simulink model "QD2_DroneStack_PID_2021a"  (R2022a)
settings: Solver=ode1  StartTime=0.0  StopTime=inf  FixedStep=1/1000  RelTol=1e-3  EnableMultiTasking=on
InitFcn:
  | Motor_Mapping_7_Inch
model workspace (MAT data in the model file):
  target_system = 1
values from neighbouring files (symbols this model uses):
  KT = [0.03616,0.117,-0.01215]    [Motor_Mapping_7_Inch.m]
  Motor_Matrix = [ 0.25   -1/(2*L_Roll)    1/(2*L_Pitch)    K_Tau/4;                  0.25   -1/(2*L_Roll)   -1/(2*L_Pitch)   -K_Tau/4;                  0.25    1/(2*L_Roll)    1/(2*L_Pitch)   -K_Tau/4;                  0.25    1/(2*L_Roll)   -1/(2*L_Pitch)    K_Tau/4]    [Motor_Mapping_7_Inch.m]
undefined symbols (not defined in the file or in its folder): _Commander, _QDrone2, _Stabilizer, datetime, HIL, lf, log_, m, n, qc_get_step_size, s, saved_data
libraries: quarc_library x94, simulink x27, simulink_extras x9
(part 2 of 4)

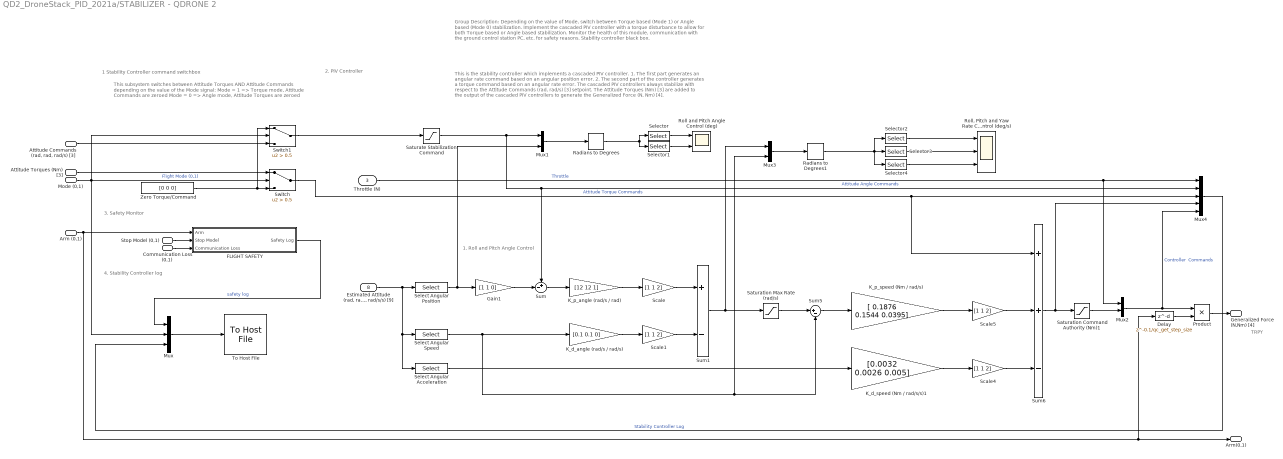
== system QD2_DroneStack_PID_2021a/STABILIZER - QDRONE 2 ==
  note: 3. Safety Monitor
  note: This subsystem switches between Attitude Torques AND Attitude Commands depending on
      | the value of the Mode signal:
      | Mode = 1	=> 		Torque mode, Attitude Commands are zeroed
      | Mode = 0	=> 		Angle mode, Attitude Torques are zeroed
  note: This is the stability controller which implements a cascaded PIV controller.
      | 1. The first part generates an angular rate command based on an angular position error.
      | 2. The second part of the controller generates a torque command based on an angular rate error.
      |
      | The cascaded PIV controllers always stabilize with respect to the Attitude Commands (rad, rad/s) [3] setpoint. The Attitude Torques (Nm) [3] are added to the output of the cascaded PIV controllers to generate the Generalized Force (N, Nm) [4].
  note: 1. Roll and Pitch Angle Control
  note: TRPY
  note: Group Description:
      |
      | Depending on the value of Mode, switch between Torque based (Mode 1) or Angle based (Mode 0) stabilization.
      | Implement the cascaded PIV controller with a torque disturbance to allow for both Torque based or Angle based stabilization.
      | Monitor the health of this module, communication with the ground control station PC, etc. for safety reasons.
      | Stability controller black box.
  note: 1 Stability Controller command switchbox
  note: 4. Stability Controller log
  note: 2. PIV Controller
  Mode (0,1) : Inport
  Stop Model (0,1) : Inport  Port=2
  Throttle (N) : Inport  Port=3
  Attitude Torques (Nm) [3] : Inport  Port=4
  "Attitude Commands (rad, rad, rad/s) [3]" : Inport  Port=5
  Arm (0,1) : Inport  Port=6
  Communication Loss (0,1) : Inport  Port=7
  "Estimated Attitude (rad, rad/s, rad/s/s) [9]" : Inport  Port=8
  Delay : Delay  DelayLength=0.1/qc_get_step_size
  FLIGHT SAFETY : Subsystem
  Gain1 : Gain  Gain=[1 1 0]
  K_d_angle (rad/s / rad/s) : Gain  Gain=[0.1 0.1 0]
  K_d_speed (Nm / rad/s/s)1 : Gain  Gain="[0.0032    0.0026     0.005]"
  K_p_angle (rad/s / rad) : Gain  Gain=[12 12 1]
  K_p_speed (Nm / rad/s) : Gain  Gain="[ 0.1876    0.1544    0.0395]"
  Mux : Mux  Inputs=3
  Mux1 : Mux  Inputs=2
  Mux2 : Mux  Inputs=2
  Mux3 : Mux  Inputs=2
  Mux4 : Mux  Inputs=5
  Product : Product
  Radians to Degrees : simulink_extras/Transformations/Radians to Degrees
  Radians to Degrees1 : simulink_extras/Transformations/Radians to Degrees
  Roll and Pitch Angle Control (deg) : Scope  NumInputPorts=2
  "Roll, Pitch and Yaw Rate Control (deg/s)" : Scope  NumInputPorts=3
  Saturate Stabilization Command : Saturate  UpperLimit=[pi/4 pi/4 10*pi/18]  LowerLimit=[-pi/4 -pi/4 -10*pi/18]
  Saturation Command Authority (Nm)1 : Saturate  UpperLimit=[1.0915 0.8984 0.0984]  LowerLimit=-[1.0915 0.8984 0.0984]
  Saturation Max Rate (rad/s) : Saturate  UpperLimit=10*pi/3*[1 1 1]  LowerLimit=-10*pi/3*[1 1 1]
  Scale{,1,4..5} (4 alike) : Gain  Gain=[1 1 2]
  Select Angular Acceleration : Selector  InputPortWidth=9  IndexOptions=Index vector (dialog)  Indices=[7:9]  OutputSizes=1
  Select Angular Speed : Selector  InputPortWidth=9  IndexOptions=Index vector (dialog)  Indices=[4:6]  OutputSizes=1
  Select Angular Position : Selector  InputPortWidth=9  IndexOptions=Index vector (dialog)  Indices=[1:3]  OutputSizes=1
  Selector : Selector  InputPortWidth=6  IndexOptions=Index vector (dialog)  Indices=[1 4]  OutputSizes=1
  Selector1 : Selector  InputPortWidth=6  IndexOptions=Index vector (dialog)  Indices=[2 5]  OutputSizes=1
  Selector2 : Selector  InputPortWidth=6  IndexOptions=Index vector (dialog)  Indices=[1 4]  OutputSizes=1
  Selector3 : Selector  InputPortWidth=6  IndexOptions=Index vector (dialog)  Indices=[2 5]  OutputSizes=1
  Selector4 : Selector  InputPortWidth=6  IndexOptions=Index vector (dialog)  Indices=[3 6]  OutputSizes=1
  Sum : Sum  Inputs=+-|
  Sum1 : Sum  Inputs=+-
  Sum5 : Sum  Inputs=|+-
  Sum6 : Sum  Inputs=++-
  Switch : Switch  Criteria=u2 > Threshold  Threshold=0.5  SaturateOnIntegerOverflow=off  InputSameDT=off
  Switch1 : Switch  Criteria=u2 > Threshold  Threshold=0.5  SaturateOnIntegerOverflow=off  InputSameDT=off
  To Host File : quarc_library/Sinks/To Host/To Host File  file_name=saved_data/%m/log_%{regexprep(char(datetime),' ','_')}_Stabilizer.mat  variable_name=stabilizer_data  decimation=1  sample_time=-1  file_format=MAT-file v.5  options=No header or footer  append=off  final_file_name=saved_data/QD2_DroneStack_PID_2021a/log_20-Nov-2026_20-05-50_Stabilizer.mat  bitrate=2000000
  Zero Torque/Command : Constant  Value=[0 0 0]
  Generalized Force (N,Nm) [4] : Outport  VectorParamsAs1DForOutWhenUnconnected=off
  Arm(0,1) : Outport  Port=2  VectorParamsAs1DForOutWhenUnconnected=off
  wires:
  Scale1/1 -> Sum1/2
  Scale/1 -> Sum1/1
  Delay/1 -> Product/2
  Zero Torque/Command/1 -> Switch1/1, Switch/3
  Attitude Torques (Nm) [3]/1 -> Switch/1
  "Attitude Commands (rad, rad, rad/s) [3]"/1 -> Switch1/3
  Radians to Degrees/1 -> Selector1/1, Selector/1
  K_d_angle (rad/s / rad/s)/1 -> Scale1/1
  Selector2/1 -> "Roll, Pitch and Yaw Rate Control (deg/s)"/1
  Selector/1 -> Roll and Pitch Angle Control (deg)/1
  Select Angular Speed/1 -> Mux3/2, Sum5/2, K_d_angle (rad/s / rad/s)/1
  K_p_angle (rad/s / rad)/1 -> Scale/1
  Selector4/1 -> "Roll, Pitch and Yaw Rate Control (deg/s)"/3
  Switch1/1 -> Saturate Stabilization Command/1
  Gain1/1 -> Sum/2
  Selector3/1 -> "Roll, Pitch and Yaw Rate Control (deg/s)"/2
  Mux1/1 -> Radians to Degrees/1
  "Estimated Attitude (rad, rad/s, rad/s/s) [9]"/1 -> Select Angular Speed/1, Select Angular Acceleration/1, Select Angular Position/1
  Radians to Degrees1/1 -> Selector3/1, Selector4/1, Selector2/1
  Switch/1 -> Sum6/1, Mux4/3  "Attitude Torque Commands"
  Selector1/1 -> Roll and Pitch Angle Control (deg)/2
  Throttle (N)/1 -> Mux4/1, Mux2/1  "Throttle"
  Select Angular Position/1 -> Mux1/2, Gain1/1
  Mux2/1 -> Product/1, Mux4/5  "Controller  Commands"
  Saturate Stabilization Command/1 -> Mux4/2, Sum/1, Mux1/1  "Attitude Angle Commands"
  Sum1/1 -> Mux3/1, Saturation Max Rate (rad/s)/1
  Mux3/1 -> Radians to Degrees1/1
  Arm (0,1)/1 -> FLIGHT SAFETY/1(Arm), Delay/1, Arm(0,1)/1
  Sum/1 -> K_p_angle (rad/s / rad)/1
  FLIGHT SAFETY/1(Safety Log) -> Mux/1  "safety log"
  Mode (0,1)/1 -> Mux/2, Switch1/2, Switch/2  "Flight Mode (0,1)"
  Mux4/1 -> Mux/3  "Stability Controller Log"
  Mux/1 -> To Host File/1
  Communication Loss (0,1)/1 -> FLIGHT SAFETY/3(Communication Loss)
  Stop Model (0,1)/1 -> FLIGHT SAFETY/2(Stop Model)
  Product/1 -> Generalized Force (N,Nm) [4]/1
  Saturation Max Rate (rad/s)/1 -> Sum5/1
  Sum5/1 -> K_p_speed (Nm / rad/s)/1
  K_p_speed (Nm / rad/s)/1 -> Scale5/1
  K_d_speed (Nm / rad/s/s)1/1 -> Scale4/1
  Scale4/1 -> Sum6/3
  Select Angular Acceleration/1 -> K_d_speed (Nm / rad/s/s)1/1
  Sum6/1 -> Mux4/4, Saturation Command Authority (Nm)1/1
  Saturation Command Authority (Nm)1/1 -> Mux2/2
  Scale5/1 -> Sum6/2

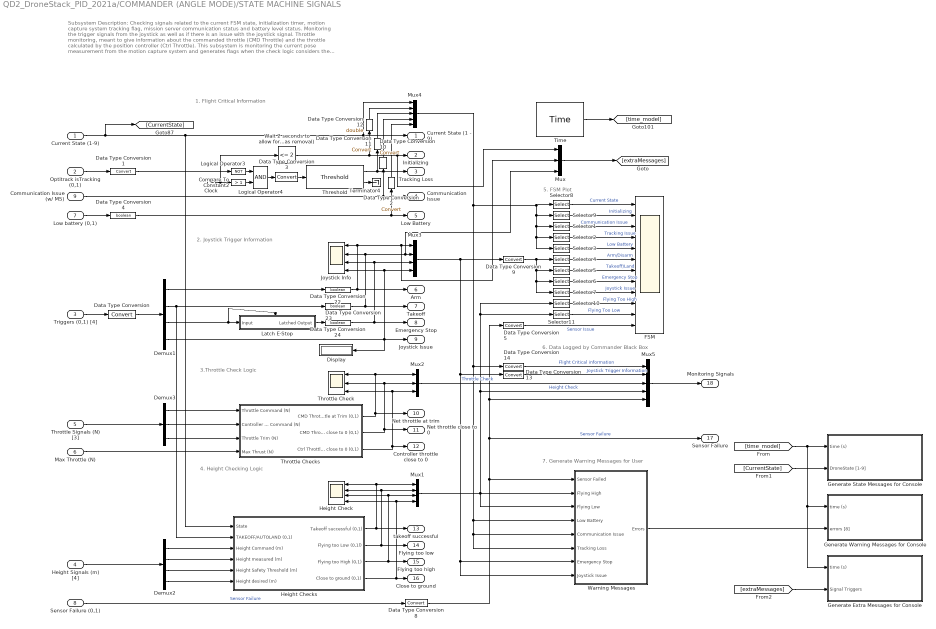
== system QD2_DroneStack_PID_2021a/COMMANDER (ANGLE MODE)/STATE MACHINE SIGNALS ==
  note: Subsystem Description:
      | Checking signals related to the current FSM state, initialization timer, motion capture system tracking flag, mission server communication status and battery level status.
      | Monitoring the trigger signals from the joystick as well as if there is an issue with the joystick signal.
      | Throttle monitoring, meant to give information about the commanded throttle (CMD Throttle) and the throttle calculated by the position controller (Ctrl Throttle).
      | This subsystem is monitoring the current pose measurement from the motion capture system and generates flags when the check logic considers the QDrone flying to close to ground, too high or too low as well as generate a successful take off flag.
      | A subset of the FSM monitoring signals are shown using this scope. These signals are what Quanser considers importnat for flight.
      | FSM signals sent to the blackbox for post flight monitoring.
      | Error message generation based on flags generated by the FSM signal checks.
  note: 7. Generate Warning Messages for User
  note: 5. FSM Plot
  note: 6. Data Logged by Commander Black Box
  note: 1. Flight Critical Information
  note: 2. Joystick Trigger Information
  note: 3.Throttle Check Logic
  note: 4. Height Checking Logic
  Current State (1-9) : Inport
  "Optitrack isTracking (0,1)  " : Inport  Port=2
  Triggers (0,1) [4] : Inport  Port=3
  Height Signals (m) [4] : Inport  Port=4
  Throttle Signals (N) [3] : Inport  Port=5
  "Max Throttle (N) " : Inport  Port=6
  Low battery (0,1) : Inport  Port=7
  Sensor Failure (0,1) : Inport  Port=8
  Communication Issue (w/ MS) : Inport  Port=9
  Clock : Clock
  Compare To Constant2 : simulink/Logic and Bit Operations/Compare To Constant  relop=>  const=1  OutDataTypeStr=boolean
  Data Type Conversion{,1..3,5,8..11,13..14} (11 alike) : DataTypeConversion  SaturateOnIntegerOverflow=off  RndMeth=Floor
  Data Type Conversion12 : DataTypeConversion  OutDataTypeStr=double  SaturateOnIntegerOverflow=off  RndMeth=Floor
  Data Type Conversion{4,22..24} (4 alike) : DataTypeConversion  OutDataTypeStr=boolean  SaturateOnIntegerOverflow=off  RndMeth=Floor
  Demux1 : Demux  Outputs=[1 1 1 1]
  Demux2 : Demux
  Demux3 : Demux  Outputs=3
  Display : Display
  FSM : Scope  NumInputPorts=12
  Generate Extra Messages for Console : Subsystem
  Generate State Messages for Console : Subsystem
  Generate Warning Messages for Console : Subsystem
  "Height Check " : Scope  NumInputPorts=4
  Height Checks : Subsystem
  Joystick Info : Scope  NumInputPorts=4
  Latch E-Stop : Subsystem  TreatAsAtomicUnit=on
  Logical Operator3 : Logic  Operator=NOT  AllPortsSameDT=off  OutDataTypeStr=boolean
  Logical Operator4 : Logic  AllPortsSameDT=off  OutDataTypeStr=boolean
  Mux : Mux  Inputs=3
  Mux1 : Mux  Inputs=[1 1 1 1]
  Mux2 : Mux  Inputs=[1 1 1]
  Mux3 : Mux  Inputs=[1 1 1 1]
  Mux4 : Mux  Inputs=[1 1 1 1 1]
  Mux5 : Mux  Inputs=[5 4 3 4 1]
  Selector1 : Selector  InputPortWidth=5  IndexOptions=Index vector (dialog)  Indices=4  OutputSizes=1
  Selector10 : Selector  InputPortWidth=4  IndexOptions=Index vector (dialog)  Indices=3  OutputSizes=1
  Selector11 : Selector  InputPortWidth=4  IndexOptions=Index vector (dialog)  Indices=2  OutputSizes=1
  Selector2 : Selector  InputPortWidth=5  IndexOptions=Index vector (dialog)  Indices=3  OutputSizes=1
  Selector3 : Selector  InputPortWidth=5  IndexOptions=Index vector (dialog)  Indices=5  OutputSizes=1
  Selector4 : Selector  InputPortWidth=4  IndexOptions=Index vector (dialog)  Indices=1  OutputSizes=1
  Selector5 : Selector  InputPortWidth=4  IndexOptions=Index vector (dialog)  Indices=2  OutputSizes=1
  Selector6 : Selector  InputPortWidth=4  IndexOptions=Index vector (dialog)  Indices=3  OutputSizes=1
  Selector7 : Selector  InputPortWidth=4  IndexOptions=Index vector (dialog)  Indices=4  OutputSizes=1
  Selector8 : Selector  InputPortWidth=5  IndexOptions=Index vector (dialog)  Indices=1  OutputSizes=1
  Selector9 : Selector  InputPortWidth=5  IndexOptions=Index vector (dialog)  Indices=2  OutputSizes=1
  Terminator4 : Terminator
  Threshold : quarc_library/Discontinuities/Threshold  operator=>=  param_src=Specify via dialog  threshold=0.5  duration=0.2
      settings: SourceProductName=QUARC Targets
  Throttle Check : Scope  NumInputPorts=3
  Throttle Checks : Subsystem
  Time : quarc_library/Sources/Time/Time  time_source=Wall clock  sample_time=qc_get_step_size
  "Wait 2 seconds to allow for initialization (e.g., bias removal)" : simulink/Logic and Bit Operations/Compare To Constant  relop=<=  const=2  OutDataTypeStr=boolean
  Warning Messages : Subsystem
  "Current State (1 - 9)  " : Outport  VectorParamsAs1DForOutWhenUnconnected=off
  Initializing : Outport  Port=2  VectorParamsAs1DForOutWhenUnconnected=off
  Tracking Loss : Outport  Port=3  VectorParamsAs1DForOutWhenUnconnected=off
  Communication Issue : Outport  Port=4  VectorParamsAs1DForOutWhenUnconnected=off
  Low Battery : Outport  Port=5  VectorParamsAs1DForOutWhenUnconnected=off
  Arm : Outport  Port=6  VectorParamsAs1DForOutWhenUnconnected=off
  Takeoff : Outport  Port=7  VectorParamsAs1DForOutWhenUnconnected=off
  Emergency Stop : Outport  Port=8  VectorParamsAs1DForOutWhenUnconnected=off
  "Joystick Issue " : Outport  Port=9  VectorParamsAs1DForOutWhenUnconnected=off
  Net throttle at trim : Outport  Port=10  VectorParamsAs1DForOutWhenUnconnected=off
  Net throttle close to 0 : Outport  Port=11  VectorParamsAs1DForOutWhenUnconnected=off
  Controller throttle close to 0 : Outport  Port=12  VectorParamsAs1DForOutWhenUnconnected=off
  takeoff successful : Outport  Port=13  VectorParamsAs1DForOutWhenUnconnected=off
  Flying too low : Outport  Port=14  VectorParamsAs1DForOutWhenUnconnected=off
  Flying too high : Outport  Port=15  VectorParamsAs1DForOutWhenUnconnected=off
  Close to ground : Outport  Port=16  VectorParamsAs1DForOutWhenUnconnected=off
  "  Sensor Failure" : Outport  Port=17  VectorParamsAs1DForOutWhenUnconnected=off
  Monitoring Signals : Outport  Port=18  VectorParamsAs1DForOutWhenUnconnected=off
  wires:
  Triggers (0,1) [4]/1 -> Data Type Conversion/1
  Demux2/1 -> Height Checks/3(Height Command (m))
  Demux3/1 -> Throttle Checks/1(Throttle Command (N))
  Height Signals (m) [4]/1 -> Demux2/1
  Demux2/4 -> Height Checks/6(Height desired (m))
  Throttle Signals (N) [3]/1 -> Demux3/1
  Demux1/1 -> Data Type Conversion22/1
  Throttle Checks/2(CMD Throttle close to 0 (0,1)) -> Mux2/2, Throttle Check/2, Net throttle close to 0/1
  Height Checks/1(Takeoff successful (0,1)) -> takeoff successful/1, "Height Check "/1, Mux1/1
  Demux2/3 -> Height Checks/5(Height Safety Threshold (m))
  Demux1/2 -> Data Type Conversion23/1, Height Checks/2(TAKEOFF/AUTOLAND (0,1))
  Demux2/2 -> Height Checks/4(Height measured (m))
  Demux3/2 -> Throttle Checks/2(Controller Throttle Command (N))
  Demux3/3 -> Throttle Checks/3(Throttle Trim (N))
  Throttle Checks/1(CMD Throttle at Trim (0,1)) -> Net throttle at trim/1, Mux2/1, Throttle Check/1
  Height Checks/3(Flying too High (0,1)) -> Mux1/3, "Height Check "/3, Flying too high/1
  Height Checks/4(Close to ground (0,1)) -> "Height Check "/4, Mux1/4, Close to ground/1
  Data Type Conversion/1 -> Demux1/1
  Low battery (0,1)/1 -> Data Type Conversion4/1
  Height Checks/2(Flying too Low (0,1l)) -> Flying too low/1, Mux1/2, "Height Check "/2
  Sensor Failure (0,1)/1 -> Data Type Conversion8/1  "Sensor Failure"
  Data Type Conversion1/1 -> Logical Operator3/1
  Data Type Conversion3/1 -> Threshold/1
  Compare To Constant2/1 -> Logical Operator4/2
  Clock/1 -> "Wait 2 seconds to allow for initialization (e.g., bias removal)"/1, Compare To Constant2/1
  Logical Operator4/1 -> Data Type Conversion3/1
  Threshold/2 -> Terminator4/1
  Logical Operator3/1 -> Logical Operator4/1
  "Optitrack isTracking (0,1)  "/1 -> Data Type Conversion1/1
  Latch E-Stop/1(Latched Output) -> Data Type Conversion24/1
  Demux1/3 -> Latch E-Stop/1(Input), Latch E-Stop/Trigger
  Selector9/1 -> FSM/2  "Initializing"
  Selector1/1 -> FSM/3  "Communication Issue"
  Selector2/1 -> FSM/4  "Tracking Issue"
  Selector3/1 -> FSM/5  "Low Battery"
  Selector4/1 -> FSM/6  "Arm/Disarm"
  Selector5/1 -> FSM/7  "Takeoff/Land"
  Selector6/1 -> FSM/8  "Emergency Stop"
  Selector7/1 -> FSM/9  "Joystick Issue"
  Data Type Conversion5/1 -> FSM/12  "Sensor Issue"
  Selector10/1 -> FSM/10  "Flying Too High"
  Selector11/1 -> FSM/11  "Flying Too Low"
  Data Type Conversion24/1 -> Joystick Info/3, Mux3/3, Emergency Stop/1
  Data Type Conversion23/1 -> Joystick Info/2, Mux/3, Mux3/2, Takeoff/1
  Data Type Conversion22/1 -> Joystick Info/1, Mux/2, Mux3/1, Arm/1
  Data Type Conversion4/1 -> Low Battery/1, Data Type Conversion2/1
  Demux1/4 -> Display/1, Joystick Info/4, Mux3/4, "Joystick Issue "/1
  Communication Issue (w/ MS)/1 -> Communication Issue/1, Data Type Conversion10/1
  Threshold/1 -> Tracking Loss/1, Data Type Conversion11/1
  Mux5/1 -> Monitoring Signals/1
  Mux1/1 -> Warning Messages/3(Flying Low), Warning Messages/2(Flying High), Selector11/1, Selector10/1, Mux5/4  "Height Check"
  Mux2/1 -> Mux5/3  "Throttle Check"
  Mux3/1 -> Data Type Conversion9/1, Warning Messages/7("Emergency Stop "), Warning Messages/8(Joystick Issue), Data Type Conversion13/1
  Mux4/1 -> Warning Messages/4(Low Battery), Warning Messages/5(Communication Issue), Warning Messages/6(Tracking Loss), Data Type Conversion14/1, Selector3/1, Selector2/1, Selector1/1, Selector9/1, Selector8/1
  Throttle Checks/3(Ctrl Throttle close to 0 (0,1)) -> Mux2/3, Throttle Check/3, Controller throttle close to 0/1
  Data Type Conversion9/1 -> Selector4/1, Selector5/1, Selector7/1, Selector6/1
  Data Type Conversion8/1 -> "  Sensor Failure"/1, Data Type Conversion5/1, Mux5/5, Warning Messages/1(Sensor Failed)  "Sensor Failure"
  Current State (1-9)/1 -> [CurrentState], Mux4/1, "Current State (1 - 9)  "/1, Height Checks/1(State)
  Selector8/1 -> FSM/1  "Current State"
  Data Type Conversion2/1 -> Mux4/5
  Data Type Conversion10/1 -> Mux4/4
  Data Type Conversion11/1 -> Mux4/3
  Data Type Conversion12/1 -> Mux4/2
  Data Type Conversion13/1 -> Mux5/2  "Joystick Trigger Information"
  Data Type Conversion14/1 -> Mux5/1  "Flight Critical information"
  "Wait 2 seconds to allow for initialization (e.g., bias removal)"/1 -> Data Type Conversion12/1, Mux/1, Initializing/1
  "Max Throttle (N) "/1 -> Throttle Checks/4(Max Thrust (N))
  Time/1 -> [time_model]
  [time_model] -> Generate Warning Messages for Console/1(time (s)), Generate Extra Messages for Console/1(time (s)), Generate State Messages for Console/1(time (s))
  [CurrentState] -> Generate State Messages for Console/2(DroneState [1-9])
  Warning Messages/1(Errors) -> Generate Warning Messages for Console/2(errors [8])
  Mux/1 -> [extraMessages]
  [extraMessages] -> Generate Extra Messages for Console/2(Signal Triggers)

== system QD2_DroneStack_PID_2021a/COMMANDER (ANGLE MODE)/Signal Smoothing ==
  "High Frequency Controller Commands (N,rad, rad/s)[4]" : Inport
  Constant4 : Constant
  Constant5 : Constant  Value=100
  Mux : Mux  Inputs=2
  Second-Order Low-Pass Filter : quarc_library/Continuous/Second-Order Low-Pass Filter  params_source=External (input ports)  input_width=60  input_zeta=1  input_init=0
  Selector1 : Selector  InputPortWidth=4  IndexOptions=Index vector (dialog)  Indices=[3:4]  OutputSizes=1
  Selector3 : Selector  InputPortWidth=4  IndexOptions=Index vector (dialog)  Indices=[1:2]  OutputSizes=1
  Terminator : Terminator
  "Smoothed Controller Commands (N,rad, rad/s)[4]" : Outport
  wires:
  "High Frequency Controller Commands (N,rad, rad/s)[4]"/1 -> Selector1/1, Selector3/1
  Mux/1 -> "Smoothed Controller Commands (N,rad, rad/s)[4]"/1
  Selector1/1 -> Mux/2
  Second-Order Low-Pass Filter/1 -> Mux/1
  Selector3/1 -> Second-Order Low-Pass Filter/4, Second-Order Low-Pass Filter/1
  Constant4/1 -> Second-Order Low-Pass Filter/3
  Constant5/1 -> Second-Order Low-Pass Filter/2
  Second-Order Low-Pass Filter/2 -> Terminator/1

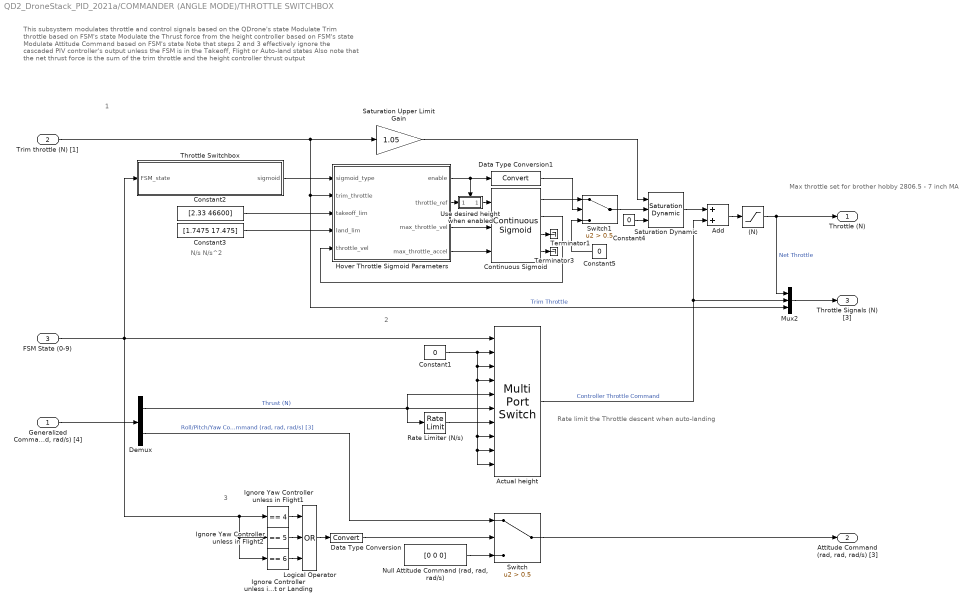
== system QD2_DroneStack_PID_2021a/COMMANDER (ANGLE MODE)/THROTTLE SWITCHBOX  ==
  note: Max throttle set for brother hobby 2806.5 - 7 inch MA
  note: 3
  note: 2
  note: 1
  note: Rate limit the Throttle descent when auto-landing
  note: This subsystem modulates throttle and control signals based on the QDrone's state
      | Modulate Trim throttle based on FSM's state
      | Modulate the Thrust force from the height controller based on FSM's state
      | Modulate Attitude Command based on FSM's state
      |
      | Note that steps 2 and 3 effectively ignore the cascaded PIV controller's output unless the FSM is in the Takeoff, Flight or Auto-land states
      | Also note that the net thrust force is the sum of the trim throttle and the height controller thrust output
  note: N/s N/s^2
  "Generalized Command (N, rad, rad, rad/s) [4]" : Inport
  Trim throttle (N) [1] : Inport  Port=2
  FSM State (0-9) : Inport  Port=3
  (N) : Saturate  UpperLimit=58  LowerLimit=0
  Actual height : MultiPortSwitch  Inputs=9  SaturateOnIntegerOverflow=off  InputSameDT=off
  Add : Sum
  Constant1 : Constant  Value=0
  Constant2 : Constant  Value=[2.33 46600]
  Constant3 : Constant  Value=[1.7475 17.475]
  Constant4 : Constant  Value=0
  Constant5 : Constant  Value=0
  Continuous Sigmoid : quarc_library/Sources/Sigmoids/Continuous Sigmoid  params_source=External (input ports)  max_velocity=2  max_acceleration=10  initial_position=0  initial_velocity=0  hold_off=0.5  input_sample_time=-1  output_sample_time=qc_get_step_size
      settings: SourceProductName=QUARC Targets
  Data Type Conversion : DataTypeConversion  SaturateOnIntegerOverflow=off  RndMeth=Floor
  Data Type Conversion1 : DataTypeConversion  SaturateOnIntegerOverflow=off  RndMeth=Floor
  Demux : Demux  Outputs=[1 3]
  Hover Throttle Sigmoid Parameters : MATLAB Function  TreatAsAtomicUnit=on
  "Ignore Controller unless in Takeoff, Flight or Landing" : simulink/Logic and Bit Operations/Compare To Constant  relop===  const=6  OutDataTypeStr=boolean
  Ignore Yaw Controller unless in Flight1 : simulink/Logic and Bit Operations/Compare To Constant  relop===  const=4  OutDataTypeStr=boolean
  Ignore Yaw Controller unless in Flight2 : simulink/Logic and Bit Operations/Compare To Constant  relop===  const=5  OutDataTypeStr=boolean
  Logical Operator : Logic  Operator=OR  Inputs=3  AllPortsSameDT=off  OutDataTypeStr=boolean
  Mux2 : Mux  Inputs=3
  "Null Attitude Command (rad, rad, rad/s)" : Constant  Value=[0 0 0]
  Rate Limiter (N/s) : RateLimiter  RisingSlewLimit=100  FallingSlewLimit=-100  SampleTimeMode=inherited
  Saturation Dynamic : simulink/Discontinuities/Saturation Dynamic  OutMin=[]  OutMax=[]  OutDataTypeStr=Inherit: Same as second input  OutDataType=fixdt(1, 16)  OutScaling=2^-10  DoSatur=off
  Saturation Upper Limit Gain : Gain  Gain=1.05
  Switch : Switch  Criteria=u2 > Threshold  Threshold=0.5  SaturateOnIntegerOverflow=off  InputSameDT=off
  Switch1 : Switch  Criteria=u2 > Threshold  Threshold=0.5  SaturateOnIntegerOverflow=off  InputSameDT=off
  Terminator1 : Terminator
  Terminator3 : Terminator
  Throttle Switchbox : MATLAB Function  TreatAsAtomicUnit=on
  Use desired height when enabled : Subsystem  TreatAsAtomicUnit=on
  Throttle (N) : Outport  VectorParamsAs1DForOutWhenUnconnected=off
  "Attitude Command (rad, rad, rad/s) [3]" : Outport  Port=2  VectorParamsAs1DForOutWhenUnconnected=off
  Throttle Signals (N) [3] : Outport  Port=3  VectorParamsAs1DForOutWhenUnconnected=off
  wires:
  Actual height/1 -> Mux2/2, Add/2  "Controller Throttle Command"
  Add/1 -> (N)/1
  (N)/1 -> Mux2/1, Throttle (N)/1  "Net Throttle"
  "Generalized Command (N, rad, rad, rad/s) [4]"/1 -> Demux/1
  Mux2/1 -> Throttle Signals (N) [3]/1
  Ignore Yaw Controller unless in Flight2/1 -> Logical Operator/2
  Data Type Conversion/1 -> Switch/2
  "Null Attitude Command (rad, rad, rad/s)"/1 -> Switch/3
  Ignore Yaw Controller unless in Flight1/1 -> Logical Operator/1
  Demux/2 -> Switch/1  "Roll/Pitch/Yaw Command (rad, rad, rad/s) [3]"
  FSM State (0-9)/1 -> Actual height/1, "Ignore Controller unless in Takeoff, Flight or Landing"/1, Ignore Yaw Controller unless in Flight2/1, Ignore Yaw Controller unless in Flight1/1, Throttle Switchbox/1(FSM_state)
  "Ignore Controller unless in Takeoff, Flight or Landing"/1 -> Logical Operator/3
  Logical Operator/1 -> Data Type Conversion/1
  Demux/1 -> Actual height/6, Rate Limiter (N/s)/1, Actual height/5  "Thrust (N)"
  Continuous Sigmoid/2 -> Hover Throttle Sigmoid Parameters/5(throttle_vel)
  Constant4/1 -> Saturation Dynamic/3
  Saturation Dynamic/1 -> Add/1
  Constant3/1 -> Hover Throttle Sigmoid Parameters/4(land_lim)
  Switch1/1 -> Saturation Dynamic/2
  Trim throttle (N) [1]/1 -> Mux2/3, Hover Throttle Sigmoid Parameters/2(trim_throttle), Saturation Upper Limit Gain/1  "Trim Throttle"
  Throttle Switchbox/1(sigmoid) -> Hover Throttle Sigmoid Parameters/1(sigmoid_type)
  Saturation Upper Limit Gain/1 -> Saturation Dynamic/1
  Constant2/1 -> Hover Throttle Sigmoid Parameters/3(takeoff_lim)
  Hover Throttle Sigmoid Parameters/4(max_throttle_accel) -> Continuous Sigmoid/3
  Continuous Sigmoid/1 -> Switch1/1
  Continuous Sigmoid/4 -> Terminator3/1
  Hover Throttle Sigmoid Parameters/3(max_throttle_vel) -> Continuous Sigmoid/2
  Data Type Conversion1/1 -> Switch1/2
  Hover Throttle Sigmoid Parameters/1(enable) -> Data Type Conversion1/1, Use desired height when enabled/Enable
  Continuous Sigmoid/3 -> Terminator1/1
  Use desired height when enabled/1(Out1) -> Continuous Sigmoid/1
  Hover Throttle Sigmoid Parameters/2(throttle_ref) -> Use desired height when enabled/1(h_d (m) [1])
  Constant5/1 -> Switch1/3
  Switch/1 -> "Attitude Command (rad, rad, rad/s) [3]"/1
  Constant1/1 -> Actual height/8, Actual height/10, Actual height/9, Actual height/4, Actual height/3, Actual height/2
  Rate Limiter (N/s)/1 -> Actual height/7

== system QD2_DroneStack_PID_2021a/Communication/Detect Communication Loss ==
  note: Stream Loss: Check if the state is 2 and error is positive (error codes are negative). Otherwise issue a communication error.
      | OR
      | Data Loss: Check if the data is stale for a while (this is required because a connected stream may publish no new data). If stale, issue a communication error.
  State : Inport
  Error : Inport  Port=2
  Data Out : Inport  Port=3
  Clock1 : Clock
  Communication Loss : Scope  NumInputPorts=2
  Data Type Conversion4 : DataTypeConversion  SaturateOnIntegerOverflow=off  RndMeth=Floor
  Grab mission server time to detect flat lines : Selector  InputPortWidth=16  IndexOptions=Index vector (dialog)  Indices=[16]  OutputSizes=1
  Logical Operator4 : Logic  Operator=OR  AllPortsSameDT=off  OutDataTypeStr=boolean
  MATLAB Function : MATLAB Function  TreatAsAtomicUnit=on
  Terminator3 : Terminator
  Terminator5 : Terminator
  Threshold1 : quarc_library/Discontinuities/Threshold  operator=>=  param_src=Specify via dialog  threshold=0.5  duration=0.1
      settings: SourceProductName=QUARC Targets
  Threshold2 : quarc_library/Discontinuities/Threshold  operator=>=  param_src=Specify via dialog  threshold=0.5  duration=0.5
      settings: SourceProductName=QUARC Targets
  Communication Issue : Outport  VectorParamsAs1DForOutWhenUnconnected=off
  wires:
  Threshold2/1 -> Communication Loss/2, Logical Operator4/2
  Logical Operator4/1 -> Data Type Conversion4/1
  Threshold1/2 -> Terminator3/1
  MATLAB Function/2(data_loss) -> Threshold2/1
  MATLAB Function/1(stream_connection_loss) -> Threshold1/1
  Clock1/1 -> MATLAB Function/1(time)
  Threshold2/2 -> Terminator5/1
  Threshold1/1 -> Communication Loss/1, Logical Operator4/1
  Grab mission server time to detect flat lines/1 -> MATLAB Function/4(ms_time)
  Data Out/1 -> Grab mission server time to detect flat lines/1
  State/1 -> MATLAB Function/2(state)
  Error/1 -> MATLAB Function/3(error)
  Data Type Conversion4/1 -> Communication Issue/1

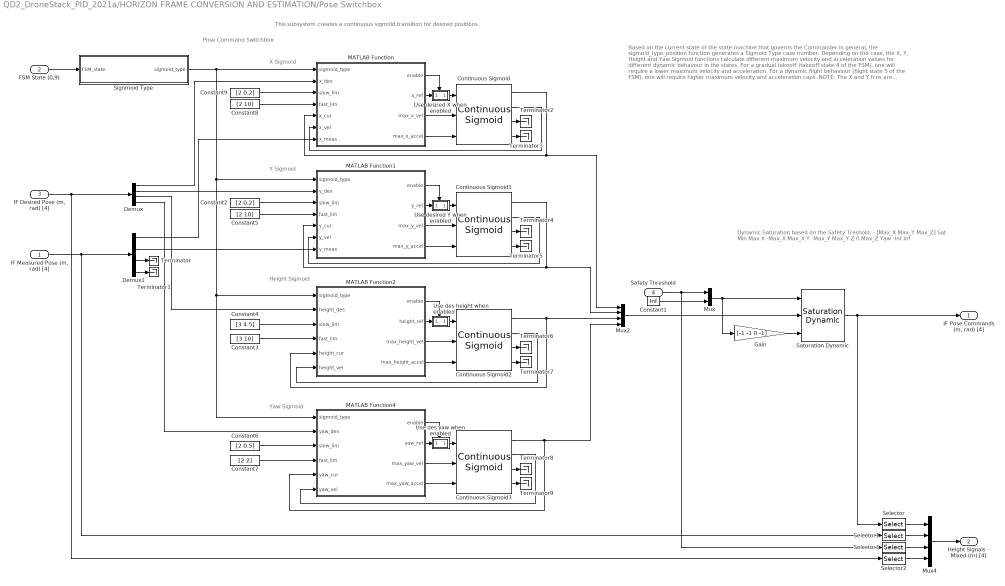
== system QD2_DroneStack_PID_2021a/HORIZON FRAME CONVERSION AND ESTIMATION/Pose Switchbox ==
  note: Dynamic Saturation based on the Safety Treshold. - [Max_X Max_Y Max_Z]
      |
      | Sat Min Max
      | X -Max_X Max_X
      | Y -Max_Y Max_Y
      | Z 0 Max_Z
      | Yaw -Inf Inf
  note: Based on the current state of the state machine that governs the Commander in general,
      | the sigmoid_type_position function generates a Sigmoid Type case number. Depending on
      | the case, the X, Y, Height and Yaw Sigmoid functions calculate different maximum velocity
      | and acceleration values for different dynamic behavour in the states.
      |
      | For a gradual takeoff (takeoff state 4 of the FSM), one will require a lower maximum velocity
      | and acceleration. For a dynamic flight behaviour (flight state 5 of the FSM), one will require
      | higher maximum velocity and acceleration caps.
      |
      | NOTE: The X and Y fcns are logically identical due to the generally symmetric X and Y behaviour.
      | The Z and Yaw fcns are different.
  note: This subsystem creates a continuous sigmoid transition for desired positions.
  note: Height Sigmoid
  note: Pose Command Switchbox
  note: X Sigmoid
  note: Yaw Sigmoid
  note: Y Sigmoid
  "IF Measured Pose (m, rad) [4]" : Inport
  FSM State (0,9) : Inport  Port=2
  "IF Desired Pose (m, rad) [4]" : Inport  Port=3
  Safety Threshold : Inport  Port=4
  Constant1 : Constant  Value=Inf
  Constant2 : Constant  Value=[2 0.2]
  Constant3 : Constant  Value=[3 10]
  Constant4 : Constant  Value=[3 4.5]
  Constant5 : Constant  Value=[2 10]
  Constant6 : Constant  Value=[2 0.5]
  Constant7 : Constant  Value=[2 2]
  Constant8 : Constant  Value=[2 10]
  Constant9 : Constant  Value=[2 0.2]
  Continuous Sigmoid{,1..3} (4 alike) : quarc_library/Sources/Sigmoids/Continuous Sigmoid  params_source=External (input ports)  max_velocity=2  max_acceleration=10  initial_position=0  initial_velocity=0  hold_off=0.5  input_sample_time=-1  output_sample_time=qc_get_step_size
      settings: SourceProductName=QUARC Targets
  Demux : Demux
  Demux1 : Demux
  Gain : Gain  Gain=[-1 -1 0 -1]
  MATLAB Function : MATLAB Function  TreatAsAtomicUnit=on
  MATLAB Function1 : MATLAB Function  TreatAsAtomicUnit=on
  MATLAB Function2 : MATLAB Function  TreatAsAtomicUnit=on
  MATLAB Function4 : MATLAB Function  TreatAsAtomicUnit=on
  Mux : Mux  Inputs=2
  Mux2 : Mux
  Mux4 : Mux
  Saturation Dynamic : simulink/Discontinuities/Saturation Dynamic  OutMin=[]  OutMax=[]  OutDataTypeStr=Inherit: Same as second input  OutDataType=fixdt(1, 16)  OutScaling=2^-10  DoSatur=off
  Selector : Selector  InputPortWidth=4  IndexOptions=Index vector (dialog)  Indices=[3]  OutputSizes=1
  Selector1 : Selector  InputPortWidth=4  IndexOptions=Index vector (dialog)  Indices=[3]  OutputSizes=1
  Selector2 : Selector  InputPortWidth=4  IndexOptions=Index vector (dialog)  Indices=[3]  OutputSizes=1
  Selector3 : Selector  InputPortWidth=3  IndexOptions=Index vector (dialog)  Indices=[3]  OutputSizes=1
  Signmoid Type : MATLAB Function  TreatAsAtomicUnit=on
  Terminator{,1..9} (10 alike) : Terminator
  Use des height when enabled : Subsystem  TreatAsAtomicUnit=on
  Use des yaw when enabled : Subsystem  TreatAsAtomicUnit=on
  Use desired X when enabled : Subsystem  TreatAsAtomicUnit=on
  Use desired Y when enabled : Subsystem  TreatAsAtomicUnit=on
  "IF Pose Commands (m, rad) [4]" : Outport  VectorParamsAs1DForOutWhenUnconnected=off
  Height Signals - Mixed (m) [4] : Outport  Port=2  VectorParamsAs1DForOutWhenUnconnected=off
  wires:
  Constant4/1 -> MATLAB Function2/3(slow_lim)
  Constant3/1 -> MATLAB Function2/4(fast_lim)
  Selector/1 -> Mux4/1
  Selector1/1 -> Mux4/2
  Selector2/1 -> Mux4/4
  Selector3/1 -> Mux4/3
  Safety Threshold/1 -> Mux/1, Selector3/1
  Mux/1 -> Saturation Dynamic/1, Gain/1
  Constant1/1 -> Mux/2
  Saturation Dynamic/1 -> "IF Pose Commands (m, rad) [4]"/1, Selector/1
  Mux2/1 -> Saturation Dynamic/2
  Mux4/1 -> Height Signals - Mixed (m) [4]/1
  Gain/1 -> Saturation Dynamic/3
  Demux/2 -> MATLAB Function1/2(y_des)
  Use desired Y when enabled/1(Out1) -> Continuous Sigmoid1/1
  Use desired X when enabled/1(Out1) -> Continuous Sigmoid/1
  MATLAB Function2/3(max_height_vel) -> Continuous Sigmoid2/2
  Continuous Sigmoid3/3 -> Terminator8/1
  Demux1/4 -> Terminator1/1
  MATLAB Function4/1(enable) -> Use des yaw when enabled/Enable
  Use des yaw when enabled/1(Out1) -> Continuous Sigmoid3/1
  Continuous Sigmoid1/2 -> MATLAB Function1/6(y_vel)
  Constant2/1 -> MATLAB Function1/3(slow_lim)
  Constant6/1 -> MATLAB Function4/3(slow_lim)
  Demux1/1 -> MATLAB Function/7(x_meas)
  MATLAB Function1/2(y_ref) -> Use desired Y when enabled/1(h_d (m) [1])
  Demux/3 -> MATLAB Function2/2(height_des)
  Constant7/1 -> MATLAB Function4/4(fast_lim)
  Continuous Sigmoid1/4 -> Terminator5/1
  MATLAB Function1/1(enable) -> Use desired Y when enabled/Enable
  Continuous Sigmoid2/4 -> Terminator7/1
  Demux1/3 -> Terminator/1
  Signmoid Type/1(sigmoid_type) -> MATLAB Function/1(sigmoid_type), MATLAB Function1/1(sigmoid_type), MATLAB Function2/1(sigmoid_type), MATLAB Function4/1(sigmoid_type)
  MATLAB Function/3(max_x_vel) -> Continuous Sigmoid/2
  MATLAB Function2/1(enable) -> Use des height when enabled/Enable
  Constant9/1 -> MATLAB Function/3(slow_lim)
  Continuous Sigmoid2/2 -> MATLAB Function2/6(height_vel)
  Continuous Sigmoid1/1 -> MATLAB Function1/5(y_cur), Mux2/2
  MATLAB Function4/4(max_yaw_accel) -> Continuous Sigmoid3/3
  Demux/1 -> MATLAB Function/2(x_des)
  MATLAB Function1/3(max_y_vel) -> Continuous Sigmoid1/2
  Continuous Sigmoid3/2 -> MATLAB Function4/6(yaw_vel)
  MATLAB Function2/2(height_ref) -> Use des height when enabled/1(h_d (m) [1])
  MATLAB Function/4(max_x_accel) -> Continuous Sigmoid/3
  Use des height when enabled/1(Out1) -> Continuous Sigmoid2/1
  Continuous Sigmoid2/3 -> Terminator6/1
  Demux/4 -> MATLAB Function4/2(yaw_des)
  MATLAB Function1/4(max_y_accel) -> Continuous Sigmoid1/3
  MATLAB Function/1(enable) -> Use desired X when enabled/Enable
  Continuous Sigmoid3/4 -> Terminator9/1
  MATLAB Function4/2(yaw_ref) -> Use des yaw when enabled/1(h_d (m) [1])
  FSM State (0,9)/1 -> Signmoid Type/1(FSM_state)
  MATLAB Function2/4(max_height_accel) -> Continuous Sigmoid2/3
  Continuous Sigmoid/4 -> Terminator3/1
  Continuous Sigmoid/3 -> Terminator2/1
  Continuous Sigmoid/1 -> MATLAB Function/5(x_cur), Mux2/1
  Continuous Sigmoid/2 -> MATLAB Function/6(x_vel)
  MATLAB Function/2(x_ref) -> Use desired X when enabled/1(h_d (m) [1])
  Continuous Sigmoid3/1 -> MATLAB Function4/5(yaw_cur), Mux2/4
  MATLAB Function4/3(max_yaw_vel) -> Continuous Sigmoid3/2
  Continuous Sigmoid2/1 -> MATLAB Function2/5(height_cur), Mux2/3
  Demux1/2 -> MATLAB Function1/7(y_meas)
  Continuous Sigmoid1/3 -> Terminator4/1
  "IF Measured Pose (m, rad) [4]"/1 -> Demux1/1, Selector1/1
  "IF Desired Pose (m, rad) [4]"/1 -> Demux/1, Selector2/1
  Constant5/1 -> MATLAB Function1/4(fast_lim)
  Constant8/1 -> MATLAB Function/4(fast_lim)

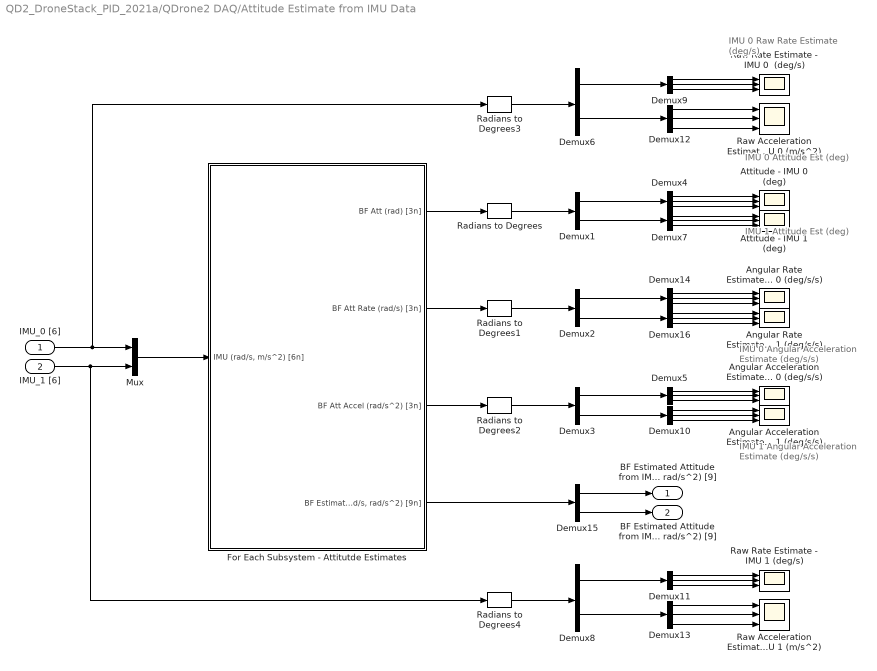
== system QD2_DroneStack_PID_2021a/QDrone2 DAQ/Attitude Estimate from IMU Data ==
  note: IMU 0
      | Attitude Est (deg)
  note: IMU 1
      | Attitude Est (deg)
  note: IMU 0
      | Angular Acceleration
      | Estimate (deg/s/s)
  note: IMU 1
      | Angular Acceleration
      | Estimate (deg/s/s)
  note: IMU 0
      | Raw Rate Estimate (deg/s)
  IMU_0 [6] : Inport
  IMU_1 [6] : Inport  Port=2
  Angular Acceleration Estimate - IMU 0 (deg/s/s) : Scope  NumInputPorts=3
  Angular Acceleration Estimate IMU 1 (deg/s/s) : Scope  NumInputPorts=3
  Angular Rate Estimate - IMU 0 (deg/s/s) : Scope  NumInputPorts=3
  Angular Rate Estimate IMU 1 (deg/s/s) : Scope  NumInputPorts=3
  Attitude - IMU 0 (deg) : Scope  NumInputPorts=3
  Attitude - IMU 1 (deg) : Scope  NumInputPorts=3
  Demux{1..3,6,8} (5 alike) : Demux  Outputs=[3, 3]
  Demux{4..5,7,9..14,16} (10 alike) : Demux  Outputs=3
  Demux15 : Demux  Outputs=[9, 9]
  For Each Subsystem - Attitutde Estimates : Subsystem  TreatAsAtomicUnit=on
  Mux : Mux  Inputs=2
  Radians to Degrees{,1..4} (5 alike) : simulink_extras/Transformations/Radians to Degrees
  Raw Acceleration Estimate - IMU 0 (m/s^2) : Scope  NumInputPorts=3
  Raw Acceleration Estimate - IMU 1 (m/s^2) : Scope  NumInputPorts=3
  Raw Rate Estimate - IMU 0  (deg/s) : Scope  NumInputPorts=3
  Raw Rate Estimate - IMU 1 (deg/s) : Scope  NumInputPorts=3
  "BF Estimated Attitude from IMU 0 (rad, rad/s, rad/s^2) [9]" : Outport
  "BF Estimated Attitude from IMU 1 (rad, rad/s, rad/s^2) [9]" : Outport  Port=2
  wires:
  IMU_0 [6]/1 -> Radians to Degrees3/1, Mux/1
  IMU_1 [6]/1 -> Radians to Degrees4/1, Mux/2
  Mux/1 -> For Each Subsystem - Attitutde Estimates/1("IMU (rad/s, m/s^2) [6n]")
  For Each Subsystem - Attitutde Estimates/4("BF Estimated Att (rad, rad/s, rad/s^2) [9n] ") -> Demux15/1
  Demux15/1 -> "BF Estimated Attitude from IMU 0 (rad, rad/s, rad/s^2) [9]"/1
  Demux15/2 -> "BF Estimated Attitude from IMU 1 (rad, rad/s, rad/s^2) [9]"/1
  For Each Subsystem - Attitutde Estimates/1(BF Att (rad) [3n]) -> Radians to Degrees/1
  Radians to Degrees/1 -> Demux1/1
  For Each Subsystem - Attitutde Estimates/2(BF Att Rate (rad/s) [3n]) -> Radians to Degrees1/1
  For Each Subsystem - Attitutde Estimates/3(BF Att Accel (rad/s^2) [3n]) -> Radians to Degrees2/1
  Radians to Degrees1/1 -> Demux2/1
  Radians to Degrees2/1 -> Demux3/1
  Demux4/3 -> Attitude - IMU 0 (deg)/3
  Demux4/1 -> Attitude - IMU 0 (deg)/1
  Demux4/2 -> Attitude - IMU 0 (deg)/2
  Demux1/1 -> Demux4/1
  Demux7/2 -> Attitude - IMU 1 (deg)/2
  Demux7/1 -> Attitude - IMU 1 (deg)/1
  Demux7/3 -> Attitude - IMU 1 (deg)/3
  Demux1/2 -> Demux7/1
  Demux5/2 -> Angular Acceleration Estimate - IMU 0 (deg/s/s)/2
  Demux5/3 -> Angular Acceleration Estimate - IMU 0 (deg/s/s)/3
  Demux5/1 -> Angular Acceleration Estimate - IMU 0 (deg/s/s)/1
  Demux3/1 -> Demux5/1
  Demux10/1 -> Angular Acceleration Estimate IMU 1 (deg/s/s)/1
  Demux10/2 -> Angular Acceleration Estimate IMU 1 (deg/s/s)/2
  Demux10/3 -> Angular Acceleration Estimate IMU 1 (deg/s/s)/3
  Demux3/2 -> Demux10/1
  Demux12/2 -> Raw Acceleration Estimate - IMU 0 (m/s^2)/2
  Demux12/3 -> Raw Acceleration Estimate - IMU 0 (m/s^2)/3
  Demux12/1 -> Raw Acceleration Estimate - IMU 0 (m/s^2)/1
  Demux8/2 -> Demux13/1
  Demux13/2 -> Raw Acceleration Estimate - IMU 1 (m/s^2)/2
  Demux13/3 -> Raw Acceleration Estimate - IMU 1 (m/s^2)/3
  Demux13/1 -> Raw Acceleration Estimate - IMU 1 (m/s^2)/1
  Demux9/2 -> Raw Rate Estimate - IMU 0  (deg/s)/2
  Demux9/1 -> Raw Rate Estimate - IMU 0  (deg/s)/1
  Demux9/3 -> Raw Rate Estimate - IMU 0  (deg/s)/3
  Demux6/2 -> Demux12/1
  Demux6/1 -> Demux9/1
  Radians to Degrees3/1 -> Demux6/1
  Radians to Degrees4/1 -> Demux8/1
  Demux11/1 -> Raw Rate Estimate - IMU 1 (deg/s)/1
  Demux11/2 -> Raw Rate Estimate - IMU 1 (deg/s)/2
  Demux11/3 -> Raw Rate Estimate - IMU 1 (deg/s)/3
  Demux8/1 -> Demux11/1
  Demux2/2 -> Demux16/1
  Demux16/3 -> Angular Rate Estimate IMU 1 (deg/s/s)/3
  Demux16/1 -> Angular Rate Estimate IMU 1 (deg/s/s)/1
  Demux16/2 -> Angular Rate Estimate IMU 1 (deg/s/s)/2
  Demux2/1 -> Demux14/1
  Demux14/2 -> Angular Rate Estimate - IMU 0 (deg/s/s)/2
  Demux14/1 -> Angular Rate Estimate - IMU 0 (deg/s/s)/1
  Demux14/3 -> Angular Rate Estimate - IMU 0 (deg/s/s)/3

== system QD2_DroneStack_PID_2021a/QDrone2 DAQ/Check Battery level ==
  Battery level : Inport
  Compare To Constant : simulink/Logic and Bit Operations/Compare To Constant  relop=<=  const=14  OutDataTypeStr=boolean
  Compare To Constant1 : simulink/Logic and Bit Operations/Compare To Constant  relop=>  const=0.5  OutDataTypeStr=boolean
  Data Type Conversion : DataTypeConversion  SaturateOnIntegerOverflow=off  RndMeth=Floor
  Data Type Conversion1 : DataTypeConversion  SaturateOnIntegerOverflow=off  RndMeth=Floor
  Logical Operator : Logic  AllPortsSameDT=off  OutDataTypeStr=boolean
  Terminator : Terminator
  Threshold : quarc_library/Discontinuities/Threshold  operator=>=  param_src=Specify via dialog  threshold=0.5  duration=0.3
      settings: SourceProductName=QUARC Targets
  Triggered Subsystem : Subsystem  TreatAsAtomicUnit=on
  Low Battery : Outport  VectorParamsAs1DForOutWhenUnconnected=off
  wires:
  Threshold/2 -> Terminator/1
  Battery level/1 -> Compare To Constant1/1, Compare To Constant/1
  Threshold/1 -> Logical Operator/2
  Logical Operator/1 -> Triggered Subsystem/Trigger
  Compare To Constant1/1 -> Logical Operator/1
  Compare To Constant/1 -> Data Type Conversion/1
  Data Type Conversion/1 -> Threshold/1
  Data Type Conversion1/1 -> Low Battery/1
  Triggered Subsystem/1(Out1) -> Data Type Conversion1/1

== system QD2_DroneStack_PID_2021a/QDrone2 DAQ/Choose Motor Telemetry ==
  Bias1 : Bias  Bias=0:3  SaturateOnIntegerOverflow=off
  Constant : Constant  Value=[0 0 0 0; 0 0 0 1; 0 0 0 0; 0 0 1 0; 0 0 0 0; 0 1 0 0; 0 0 0 0; 1 0 0 0]
  Counter Free-Running : simulink/Sources/Counter Free-Running  NumBits=3  tsamp=-1
  Gain : Gain  Gain=.7
  Selector : Selector  NumberOfDimensions=2  IndexMode=Zero-based  InputPortWidth=3  IndexOptions=Index vector (port),Select all  Indices=[1 3],1  OutputSizes=1,1
  Telemetry : Scope
  Motor telemetry : Outport
  wires:
  Gain/1 -> Bias1/1
  Bias1/1 -> Telemetry/1
  Constant/1 -> Selector/1
  Counter Free-Running/1 -> Selector/2
  Selector/1 -> Motor telemetry/1, Gain/1

== system QD2_DroneStack_PID_2021a/QDrone2 DAQ/Choose Motor Telemetry1 ==
  Channel : Inport
  Constant1 : Constant  Value=[1 0 0 0]
  Constant2 : Constant  Value=[0 1 0 0]
  Constant3 : Constant  Value=[0 0 1 0]
  Constant4 : Constant  Value=[0 0 0 1]
  Multiport Switch : MultiPortSwitch  DataPortOrder=Zero-based contiguous  Inputs=4  zeroidx=on  SaturateOnIntegerOverflow=off  InputSameDT=off
  Motor selection : Outport
  wires:
  Multiport Switch/1 -> Motor selection/1
  Constant4/1 -> Multiport Switch/5
  Constant3/1 -> Multiport Switch/4
  Constant1/1 -> Multiport Switch/2
  Constant2/1 -> Multiport Switch/3
  Channel/1 -> Multiport Switch/1

== system QD2_DroneStack_PID_2021a/QDrone2 DAQ/Sensor Failure Monitoring - IMU0 ==
  note: Check for no data condition (flat-line zero) from any of the onboard sensors
  Sensor Data (rad/s,m/s^2)  [6] : Inport
  Data Type Conversion1 : DataTypeConversion  SaturateOnIntegerOverflow=off  RndMeth=Floor
  Data Type Conversion2 : DataTypeConversion  SaturateOnIntegerOverflow=off  RndMeth=Floor
  Data Type Conversion4 : DataTypeConversion  SaturateOnIntegerOverflow=off  RndMeth=Floor
  Demux : Demux  Outputs=[3 3]
  Logical Operator : Logic  Operator=OR  Inputs=1  AllPortsSameDT=off  OutDataTypeStr=boolean
  Mux : Mux  Inputs=2
  Sensor Failure (Accelerometer) : Subsystem
  Sensor Failure (Gyroscope) : Subsystem
  IMU Failure : Outport  VectorParamsAs1DForOutWhenUnconnected=off
  wires:
  Data Type Conversion4/1 -> IMU Failure/1
  Logical Operator/1 -> Data Type Conversion4/1
  Demux/1 -> Sensor Failure (Gyroscope)/1(Sensor Input)
  Data Type Conversion1/1 -> Mux/2
  Data Type Conversion2/1 -> Mux/1
  Mux/1 -> Logical Operator/1
  Sensor Failure (Accelerometer)/1(Sensor Fault) -> Data Type Conversion1/1
  Sensor Failure (Gyroscope)/1(Sensor Fault) -> Data Type Conversion2/1
  Demux/2 -> Sensor Failure (Accelerometer)/1(Sensor Input)
  Sensor Data (rad/s,m/s^2)  [6]/1 -> Demux/1

== system QD2_DroneStack_PID_2021a/QDrone2 DAQ/Sensor Failure Monitoring - IMU1 ==
  note: Check for no data condition (flat-line zero) from any of the onboard sensors
  Sensor Data (rad/s,m/s^2)  [6] : Inport
  Data Type Conversion1 : DataTypeConversion  SaturateOnIntegerOverflow=off  RndMeth=Floor
  Data Type Conversion2 : DataTypeConversion  SaturateOnIntegerOverflow=off  RndMeth=Floor
  Data Type Conversion4 : DataTypeConversion  SaturateOnIntegerOverflow=off  RndMeth=Floor
  Demux : Demux  Outputs=[3 3]
  Logical Operator : Logic  Operator=OR  Inputs=1  AllPortsSameDT=off  OutDataTypeStr=boolean
  Mux : Mux  Inputs=2
  Sensor Failure (Accelerometer) : Subsystem
  Sensor Failure (Gyroscope) : Subsystem
  IMU Failure : Outport  VectorParamsAs1DForOutWhenUnconnected=off
  wires:
  Sensor Data (rad/s,m/s^2)  [6]/1 -> Demux/1
  Demux/2 -> Sensor Failure (Accelerometer)/1(Sensor Input)
  Sensor Failure (Gyroscope)/1(Sensor Fault) -> Data Type Conversion2/1
  Sensor Failure (Accelerometer)/1(Sensor Fault) -> Data Type Conversion1/1
  Mux/1 -> Logical Operator/1
  Data Type Conversion2/1 -> Mux/1
  Data Type Conversion1/1 -> Mux/2
  Demux/1 -> Sensor Failure (Gyroscope)/1(Sensor Input)
  Logical Operator/1 -> Data Type Conversion4/1
  Data Type Conversion4/1 -> IMU Failure/1

== system QD2_DroneStack_PID_2021a/QDrone2 DAQ/Subsystem ==
  note: PCB LED 2
  note: PCB LED 1
  E_Stop (0,1) : Inport
  "Arm(0,1) " : Inport  Port=2
  Battery_State (bool) : Inport  Port=3
  Blue : Constant  Value=[0 0 1]
  Green : Constant  Value=[0 1 0]
  MATLAB Function LED Color Assignment : MATLAB Function  TreatAsAtomicUnit=on
  Multiport Switch : MultiPortSwitch  SaturateOnIntegerOverflow=off  InputSameDT=off
  Mux : Mux  Inputs=2
  Red : Constant  Value=[1 0 0]
  LEDs(%) [6] : Outport
  wires:
  Mux/1 -> LEDs(%) [6]/1
  Multiport Switch/1 -> Mux/1, Mux/2
  Blue/1 -> Multiport Switch/4
  Green/1 -> Multiport Switch/3
  Red/1 -> Multiport Switch/2
  Battery_State (bool)/1 -> MATLAB Function LED Color Assignment/3(low_battery)
  E_Stop (0,1)/1 -> MATLAB Function LED Color Assignment/1(E_Stop)
  "Arm(0,1) "/1 -> MATLAB Function LED Color Assignment/2(Arm)
  MATLAB Function LED Color Assignment/1(value) -> Multiport Switch/1

== system QD2_DroneStack_PID_2021a/QDrone2 DAQ/Subsystem1 ==
  ESC % : Inport
  Motor command : Inport  Port=2
  Demux1 : Demux
  Demux3 : Demux
  Maintain previous value4 : Subsystem
  Mux{,1..3} (4 alike) : Mux  Inputs=2
  Selector : Selector  InputPortWidth=4  IndexOptions=Index vector (dialog)  Indices=[4 3 2 1]  OutputSizes=1
  Selector1 : Selector  InputPortWidth=4  IndexOptions=Index vector (dialog)  Indices=[4 3 2 1]  OutputSizes=1
  Out1 : Outport
  Out2 : Outport  Port=2
  Out3 : Outport  Port=3
  Out4 : Outport  Port=4
  wires:
  Motor command/1 -> Selector/1
  Demux1/2 -> Mux1/1
  Selector/1 -> Demux1/1
  Demux1/1 -> Mux/1
  Demux1/4 -> Mux3/1
  Demux1/3 -> Mux2/1
  Mux3/1 -> Out4/1
  Mux2/1 -> Out3/1
  Mux/1 -> Out1/1
  Mux1/1 -> Out2/1
  ESC %/1 -> Selector1/1
  Demux3/1 -> Mux/2
  Demux3/2 -> Mux1/2
  Demux3/3 -> Mux2/2
  Demux3/4 -> Mux3/2
  Selector1/1 -> Maintain previous value4/1(Value in)
  Maintain previous value4/1(Non 0 values) -> Demux3/1

== system QD2_DroneStack_PID_2021a/STABILIZER - QDRONE 2/FLIGHT SAFETY ==
  note: If the watchdog times out, stop the model. This will shut off the motors as well.
  note: If communication with the model supplying reference commands has been lost for some time while the drone is armed, stop the model. This will shut off the motors as well.
  note: If the model supplying reference commands triggers a STOP MODEL command, stop this model. This will shut off the motors as well.
  note: Log Computation Time. This must be less than 0.001 s
  note: Log Sample Time. This must be approximately 0.001 s
  note: Flight Safety Information
      |
      | When a warning/stop message pops up, this is the subsystem
      | that generates them.
      |
      | Monitor Sample/Computation Time
      | Stop this model
      | when Stop Model is generated
      | communication loss is detected
      | Also log the watchdog monitor output
  Arm : Inport
  Stop Model : Inport  Port=2
  Communication Loss : Inport  Port=3
  Communication : quarc_library/Discontinuities/Threshold  operator=>=  param_src=Specify via dialog  threshold=0.5  duration=1
      settings: SourceProductName=QUARC Targets
  Computation Time : quarc_library/Sources/Time/Computation Time  sample_time=qc_get_step_size  use_model=on  use_cpu_time=off
  Computation Time (s) : Scope
  Data Type Conversion1 : DataTypeConversion  SaturateOnIntegerOverflow=off  RndMeth=Floor
  Data Type Conversion3 : DataTypeConversion  OutDataTypeStr=double  SaturateOnIntegerOverflow=off  RndMeth=Floor
  Data Type Conversion4 : DataTypeConversion  SaturateOnIntegerOverflow=off  RndMeth=Floor
  Data Type Conversion5 : DataTypeConversion  SaturateOnIntegerOverflow=off  RndMeth=Floor
  HIL Watchdog : quarc_library/Data Acquisition/Generic/Watchdog/HIL Watchdog  object_name=HIL-1  timeout=0.1  sample_time=qc_get_step_size  active=off
      settings: AttributesFormatString=(%<object_name>)  SourceProductName=QUARC Targets
  Logical Operator1 : Logic  AllPortsSameDT=off  OutDataTypeStr=boolean
  Mux : Mux
  Mux1 : Mux  Inputs=2
  Sample Time : quarc_library/Sources/Time/Sample Time  Priority=-99  sample_time=qc_get_step_size
  Sample Time (s) : Scope
  Stop model : quarc_library/Discontinuities/Threshold  operator=>=  param_src=Specify via dialog  threshold=0.5  duration=0.1
      settings: SourceProductName=QUARC Targets
  Stop with Message : quarc_library/Sinks/Error Handling/Stop with Message  message_type=Fixed error message  message_icon=Information  message=QDrone Stabilizer: Commander Terminated
  Stop with Message1 : quarc_library/Sinks/Error Handling/Stop with Message  message_type=Fixed error message  message_icon=Warning  message=QDrone Stabilizer: Communication with Commander lost
  Stop with Message3 : quarc_library/Sinks/Error Handling/Stop with Message  message_type=Fixed error message  message_icon=Information  message=QDrone Stabilizer: HIL Watchdog timer expired
  Terminator : Terminator
  Terminator1 : Terminator
  Safety Log : Outport  VectorParamsAs1DForOutWhenUnconnected=off
  wires:
  Data Type Conversion5/1 -> Mux/4
  Mux1/1 -> Mux/1
  Communication Loss/1 -> Logical Operator1/1
  Data Type Conversion3/1 -> Communication/1
  Communication/1 -> Stop with Message1/1, Data Type Conversion1/1
  Arm/1 -> Logical Operator1/2
  Data Type Conversion1/1 -> Mux/3
  Logical Operator1/1 -> Data Type Conversion3/1
  Communication/2 -> Terminator1/1
  Stop Model/1 -> Stop model/1
  Stop model/1 -> Stop with Message/1, Data Type Conversion4/1
  Stop model/2 -> Terminator/1
  HIL Watchdog/1 -> Data Type Conversion5/1, Stop with Message3/1
  Data Type Conversion4/1 -> Mux/2
  Sample Time/1 -> Mux1/1, Sample Time (s)/1
  Computation Time/1 -> Mux1/2, Computation Time (s)/1
  Mux/1 -> Safety Log/1
